simulink model "Three_Stages"  (R2023a)
settings: Solver=FixedStepDiscrete  StartTime=0.0  StopTime=5000  FixedStep=1  RelTol=1e-3
values from neighbouring files (symbols this model uses):
  fw = zeros(16384, 1, 'uint32')    [test.m]
libraries: hdlsllib x27, simulink x27, etargetslib x1
(part 3 of 5)

== system Three_Stages/Subsystem5 ==
  note: // EX -> ID APSR forwarding: CMP/SUBS flags visible to branches in ID
  In2 : Inport
  In5 : Inport  Port=2
  In6 : Inport  Port=3
  In4 : Inport  Port=4
  fwd_n : Inport  Port=5
  fwd_z : Inport  Port=6
  fwd_v : Inport  Port=7
  fwd_c : Inport  Port=8
  alu_n : Inport  Port=9
  alu_z : Inport  Port=10
  alu_v : Inport  Port=11
  alu_c : Inport  Port=12
  Logical Operator : Logic  Inputs=4  AllPortsSameDT=off  OutDataTypeStr=boolean
  Logical Operator1 : Logic  Operator=NOT  AllPortsSameDT=off  OutDataTypeStr=boolean
  Switch{,1..3} (4 alike) : Switch  Criteria=u2 ~= 0  SaturateOnIntegerOverflow=off  InputSameDT=off
  id_instr8 : Outport
  id_instr9 : Outport  Port=2
  id_instr10 : Outport  Port=3
  id_instr11 : Outport  Port=4
  wires:
  alu_z/1 -> Switch/1  "ex_alu_z"
  fwd_z/1 -> Switch/3  "fwd_z"
  In2/1 -> Logical Operator/1  "ex_valid"
  In4/1 -> Logical Operator/2  "ex_s"
  In5/1 -> Logical Operator/3  "ex_cond_ok"
  In6/1 -> Logical Operator1/1  "ex_is_multi_op_raw_nf"
  Logical Operator1/1 -> Logical Operator/4
  Switch/1 -> id_instr8/1  "branch_fwd_z"
  alu_n/1 -> Switch1/1  "ex_alu_n"
  fwd_n/1 -> Switch1/3  "fwd_n"
  Switch1/1 -> id_instr9/1  "branch_fwd_n"
  alu_c/1 -> Switch2/1  "ex_alu_c"
  fwd_c/1 -> Switch2/3  "fwd_c"
  Switch2/1 -> id_instr10/1  "branch_fwd_c"
  alu_v/1 -> Switch3/1  "ex_alu_v"
  fwd_v/1 -> Switch3/3  "fwd_v"
  Switch3/1 -> id_instr11/1  "branch_fwd_v"
  Logical Operator/1 -> Switch3/2, Switch2/2, Switch1/2, Switch/2  "ex_sets_flags"

== system Three_Stages/Subsystem7 ==
  Constant1 : Constant  OutDataTypeStr=boolean
  Constant9 : Constant  OutDataTypeStr=boolean
  Switch1 : Switch  Criteria=u2 ~= 0  SaturateOnIntegerOverflow=off  InputSameDT=off
  Switch13 : Switch  Criteria=u2 ~= 0  SaturateOnIntegerOverflow=off  InputSameDT=off
  rf_we_int : Outport
  tag scope: rf_we_int=global
  wires:
  [mr_rf_we] -> Switch13/2
  Switch1/1 -> Switch13/3
  Constant9/1 -> Switch13/1
  Switch13/1 -> [rf_we_int], rf_we_int/1  "rf_we_int"
  Constant1/1 -> Switch1/1
  [wb_lo_en] -> Switch1/3
  [two_wb_d] -> Switch1/2  "two_wb_d"

== system Three_Stages/Subsystem8 ==
  Switch1 : Switch  Criteria=u2 ~= 0  SaturateOnIntegerOverflow=off  InputSameDT=off
  Switch11 : Switch  Criteria=u2 ~= 0  SaturateOnIntegerOverflow=off  InputSameDT=off
  Switch2 : Switch  Criteria=u2 ~= 0  SaturateOnIntegerOverflow=off  InputSameDT=off
  rf_we_addr_int : Outport
  tag scope: rf_we_addr_int=global
  wires:
  [mr_rf_addr] -> Switch11/1
  [mr_rf_we] -> Switch11/2
  Switch11/1 -> [rf_we_addr_int], rf_we_addr_int/1  "rf_we_addr_int"
  [ex_WB_addr] -> Switch2/3  "ex_WB_addr"
  Switch1/1 -> Switch11/3
  [two_wb_d] -> Switch1/2  "two_wb_d"
  [ex_rd_hi] -> Switch1/1
  Switch2/1 -> Switch1/3
  [ex_two_wb_active] -> Switch2/2  "ex_two_wb_active"
  [ex_rd_lo] -> Switch2/1  "ex_rd_lo"

== system Three_Stages/Subsystem9 ==
  Switch1 : Switch  Criteria=u2 ~= 0  SaturateOnIntegerOverflow=off  InputSameDT=off
  Switch10 : Switch  Criteria=u2 ~= 0  SaturateOnIntegerOverflow=off  InputSameDT=off
  rf_wdata_int : Outport
  wires:
  [mr_rf_wdata] -> Switch10/1
  [mr_rf_we] -> Switch10/2
  Switch10/1 -> rf_wdata_int/1  "rf_wdata_int"
  [rf_wdata] -> Switch1/3  "rf_wdata"
  [two_wb_d] -> Switch1/2  "two_wb_d"
  Switch1/1 -> Switch10/3  "rf_wdata_int"
  [alu_result_hi] -> Switch1/1

== system Three_Stages/i ==
  opcode : Inport
  Constant : Constant  Value=84
  Constant1 : Constant  Value=86
  Constant2 : Constant  Value=58
  Logical Operator : Logic  Operator=OR  AllPortsSameDT=off  OutDataTypeStr=boolean
  Logical Operator1 : Logic  Operator=OR  AllPortsSameDT=off  OutDataTypeStr=boolean
  Relational Operator : RelationalOperator  Operator===  OutDataTypeStr=boolean  RndMeth=Simplest  InputSameDT=off
  Relational Operator1 : RelationalOperator  Operator===  OutDataTypeStr=boolean  RndMeth=Simplest  InputSameDT=off
  Relational Operator2 : RelationalOperator  Operator===  OutDataTypeStr=boolean  RndMeth=Simplest  InputSameDT=off
  Out3 : Outport
  wires:
  Constant/1 -> Relational Operator/2
  Relational Operator/1 -> Logical Operator/1
  Constant1/1 -> Relational Operator1/2
  Relational Operator1/1 -> Logical Operator/2
  Logical Operator/1 -> Logical Operator1/1  "is_adr"
  Constant2/1 -> Relational Operator2/2
  Relational Operator2/1 -> Logical Operator1/2  "is_ldr_lit"
  opcode/1 -> Relational Operator2/1, Relational Operator1/1, Relational Operator/1  "ex_opcode"
  Logical Operator1/1 -> Out3/1  "needs_pc"

== system Three_Stages/id_pc_val2 ==
  In1 : Inport
  In4 : Inport  Port=2
  In5 : Inport  Port=3
  Add : Sum
  Add1 : Sum
  Constant : Constant  Value=4
  Constant1 : Constant  Value=2
  Switch1 : Switch  Criteria=u2 ~= 0  SaturateOnIntegerOverflow=off  InputSameDT=off
  Switch2 : Switch  Criteria=u2 ~= 0  SaturateOnIntegerOverflow=off  InputSameDT=off
  Out1 : Outport
  wires:
  Constant/1 -> Add/2
  Add/1 -> Switch1/1  "pc_plus4"
  Constant1/1 -> Add1/2
  In1/1 -> Switch2/3, Add/1, Add1/1  "pc_addr"
  Add1/1 -> Switch1/3  "pc_plus2"
  In4/1 -> Switch1/2  "pf_width"
  Switch1/1 -> Switch2/1  "pc_inc"
  In5/1 -> Switch2/2  "pf_pop_valid"
  Switch2/1 -> Out1/1  "next_pc"

== system Three_Stages/memory ==
  read_addr : Inport
  write_addr : Inport  Port=2
  read_en : Inport  Port=3
  write_en : Inport  Port=4
  write_data : Inport  Port=5
  instr_addr : Inport  Port=6
  Constant : Constant  Value=fw
  MATLAB Function1 : MATLAB Function  TreatAsAtomicUnit=on
  instr_data : Outport  OutDataTypeStr=uint32
  read_data : Outport  Port=2
  wires:
  [rst_n] -> MATLAB Function1/1(rst_n)
  read_addr/1 -> MATLAB Function1/6(read_addr)
  write_en/1 -> MATLAB Function1/2(write_en)
  read_en/1 -> MATLAB Function1/5(read_en)
  write_data/1 -> MATLAB Function1/4(write_data)
  write_addr/1 -> MATLAB Function1/3(write_addr)
  instr_addr/1 -> MATLAB Function1/7(instr_addr)
  MATLAB Function1/1(read_data) -> read_data/1  "read_data"
  MATLAB Function1/2(instr_data) -> instr_data/1  "instr_data"
  Constant/1 -> MATLAB Function1/8(fw_init)

== system Three_Stages/ALU/REV16 ==
  u : Inport
  Bit Slice2 : hdlsllib/Logic and Bit Operations/Bit Slice  lidx=7  ridx=0
  Bit Slice3 : hdlsllib/Logic and Bit Operations/Bit Slice  lidx=15  ridx=8
  Bit Slice4 : hdlsllib/Logic and Bit Operations/Bit Slice  lidx=23  ridx=16
  Bit Slice5 : hdlsllib/Logic and Bit Operations/Bit Slice  lidx=31  ridx=24
  Bitwise Operator10 : simulink/Logic and Bit Operations/Bitwise Operator  logicop=OR  UseBitMask=off  NumInputPorts=2  BitMask=bin2dec('11011001')  BitMaskRealWorld=Stored Integer
  Bitwise Operator11 : simulink/Logic and Bit Operations/Bitwise Operator  logicop=OR  UseBitMask=off  NumInputPorts=2  BitMask=bin2dec('11011001')  BitMaskRealWorld=Stored Integer
  Bitwise Operator9 : simulink/Logic and Bit Operations/Bitwise Operator  logicop=OR  UseBitMask=off  NumInputPorts=2  BitMask=bin2dec('11011001')  BitMaskRealWorld=Stored Integer
  Shift Arithmetic3 : ArithShift  BitShiftNumber=8  BitShiftDirection=Left
  Shift Arithmetic4 : ArithShift  BitShiftNumber=8  BitShiftDirection=Right
  Shift Arithmetic5 : ArithShift  BitShiftNumber=8  BitShiftDirection=Left
  Shift Arithmetic6 : ArithShift  BitShiftNumber=8  BitShiftDirection=Right
  REV16 : Outport
  wires:
  Bitwise Operator10/1 -> Bitwise Operator11/2
  Shift Arithmetic4/1 -> Bitwise Operator9/2
  Bit Slice3/1 -> Shift Arithmetic4/1
  Bit Slice2/1 -> Shift Arithmetic3/1
  u/1 -> Bit Slice5/1, Bit Slice4/1, Bit Slice3/1, Bit Slice2/1
  Bit Slice4/1 -> Shift Arithmetic5/1
  Shift Arithmetic3/1 -> Bitwise Operator9/1
  Shift Arithmetic6/1 -> Bitwise Operator10/2
  Bit Slice5/1 -> Shift Arithmetic6/1
  Shift Arithmetic5/1 -> Bitwise Operator10/1
  Bitwise Operator9/1 -> Bitwise Operator11/1
  Bitwise Operator11/1 -> REV16/1  "REV16"

== system Three_Stages/ALU/Subsystem ==
  alu_a : Inport
  Bit Slice : hdlsllib/Logic and Bit Operations/Bit Slice  lidx=7  ridx=0
  Bit Slice1 : hdlsllib/Logic and Bit Operations/Bit Slice  lidx=15  ridx=8
  Bitwise Operator11 : simulink/Logic and Bit Operations/Bitwise Operator  logicop=OR  UseBitMask=off  NumInputPorts=2  BitMask=bin2dec('11011001')  BitMaskRealWorld=Stored Integer
  Data Type Conversion1 : DataTypeConversion  OutDataTypeStr=int32  SaturateOnIntegerOverflow=off  RndMeth=Floor
  Data Type Conversion2 : DataTypeConversion  OutDataTypeStr=uint32  SaturateOnIntegerOverflow=off  RndMeth=Floor
  Data Type Conversion6 : DataTypeConversion  OutDataTypeStr=int16  SaturateOnIntegerOverflow=off  RndMeth=Floor
  Shift Arithmetic1 : ArithShift  BitShiftNumber=8  BitShiftDirection=Right
  Shift Arithmetic3 : ArithShift  BitShiftNumber=8  BitShiftDirection=Left
  Out1 : Outport
  wires:
  Bit Slice/1 -> Shift Arithmetic3/1
  Bit Slice1/1 -> Shift Arithmetic1/1
  Shift Arithmetic3/1 -> Bitwise Operator11/1
  Shift Arithmetic1/1 -> Bitwise Operator11/2
  Bitwise Operator11/1 -> Data Type Conversion6/1
  Data Type Conversion6/1 -> Data Type Conversion1/1
  Data Type Conversion1/1 -> Data Type Conversion2/1
  Data Type Conversion2/1 -> Out1/1  "REVSH"
  alu_a/1 -> Bit Slice1/1, Bit Slice/1

== system Three_Stages/ALU/Subsystem1 ==
  alu_a : Inport
  alu_b : Inport  Port=2
  Bitwise Operator1 : simulink/Logic and Bit Operations/Bitwise Operator  logicop=OR  UseBitMask=on  BitMask=0x0000FFFF  BitMaskRealWorld=Stored Integer
  Bitwise Operator2 : simulink/Logic and Bit Operations/Bitwise Operator  logicop=OR  UseBitMask=on  BitMask=0x0000FFFF  BitMaskRealWorld=Stored Integer
  Bitwise Operator3 : simulink/Logic and Bit Operations/Bitwise Operator  logicop=OR  UseBitMask=off  NumInputPorts=2  BitMask=bin2dec('11011001')  BitMaskRealWorld=Stored Integer
  Shift Arithmetic2 : ArithShift  BitShiftNumber=16  BitShiftDirection=Left
  Out1 : Outport
  wires:
  Bitwise Operator3/1 -> Out1/1  "REVSH"
  alu_a/1 -> Bitwise Operator1/1
  Bitwise Operator1/1 -> Bitwise Operator3/1  "lo_keep"
  Bitwise Operator2/1 -> Shift Arithmetic2/1  "imm_lo"
  Shift Arithmetic2/1 -> Bitwise Operator3/2
  alu_b/1 -> Bitwise Operator2/1

== system Three_Stages/ALU/Subsystem2 ==
  In1 : Inport
  In2 : Inport  Port=2
  "alu_acc " : Inport  Port=3
  Add6 : Sum  AccumDataTypeStr=uint64  OutDataTypeStr=uint32
  Data Type Conversion10 : DataTypeConversion  OutDataTypeStr=uint32  SaturateOnIntegerOverflow=off  RndMeth=Floor
  Data Type Conversion9 : DataTypeConversion  OutDataTypeStr=uint64  SaturateOnIntegerOverflow=off  RndMeth=Floor
  Product1 : Product  OutDataTypeStr=uint64
  MLA : Outport
  wires:
  In2/1 -> Product1/2
  Product1/1 -> Add6/1  "prod64"
  Data Type Conversion9/1 -> Add6/2  "acc64"
  Data Type Conversion10/1 -> MLA/1  "MLA"
  "alu_acc "/1 -> Data Type Conversion9/1  "alu_acc"
  Add6/1 -> Data Type Conversion10/1  "sum64"
  In1/1 -> Product1/1

== system Three_Stages/ALU/Subsystem3 ==
  alu_a : Inport
  alu_b : Inport  Port=2
  "alu_acc " : Inport  Port=3
  Add6 : Sum  Inputs=+-  AccumDataTypeStr=uint64  OutDataTypeStr=uint32
  Data Type Conversion10 : DataTypeConversion  OutDataTypeStr=uint32  SaturateOnIntegerOverflow=off  RndMeth=Floor
  Data Type Conversion9 : DataTypeConversion  OutDataTypeStr=uint64  SaturateOnIntegerOverflow=off  RndMeth=Floor
  Product1 : Product  OutDataTypeStr=uint64
  MLS : Outport
  wires:
  alu_b/1 -> Product1/2
  Product1/1 -> Add6/2  "prod64"
  Data Type Conversion9/1 -> Add6/1  "acc64"
  Data Type Conversion10/1 -> MLS/1  "MLA"
  "alu_acc "/1 -> Data Type Conversion9/1  "alu_acc"
  Add6/1 -> Data Type Conversion10/1  "sum64"
  alu_a/1 -> Product1/1

== system Three_Stages/ALU/Subsystem4 ==
  alu_a : Inport
  alu_b : Inport  Port=2
  Bit Slice1 : hdlsllib/Logic and Bit Operations/Bit Slice  lidx=31  ridx=0
  Bit Slice2 : hdlsllib/Logic and Bit Operations/Bit Slice  lidx=63  ridx=32
  Data Type Conversion1 : DataTypeConversion  OutDataTypeStr=uint32  SaturateOnIntegerOverflow=off  RndMeth=Floor
  Data Type Conversion10 : DataTypeConversion  OutDataTypeStr=uint32  SaturateOnIntegerOverflow=off  RndMeth=Floor
  Product1 : Product  OutDataTypeStr=uint64
  MLS : Outport
  MLS1 : Outport  Port=2
  wires:
  alu_b/1 -> Product1/2
  Data Type Conversion10/1 -> MLS/1  "RdLo"
  alu_a/1 -> Product1/1
  Product1/1 -> Bit Slice2/1, Bit Slice1/1  "prod64"
  Bit Slice1/1 -> Data Type Conversion10/1  "result_lo"
  Bit Slice2/1 -> Data Type Conversion1/1  "result_hi"
  Data Type Conversion1/1 -> MLS1/1  "RdHi"

== system Three_Stages/ALU/Subsystem5 ==
  alu_a : Inport
  alu_b : Inport  Port=2
  Bit Slice1 : hdlsllib/Logic and Bit Operations/Bit Slice  lidx=31  ridx=0
  Bit Slice2 : hdlsllib/Logic and Bit Operations/Bit Slice  lidx=63  ridx=32
  Data Type Conversion1 : DataTypeConversion  OutDataTypeStr=uint32  SaturateOnIntegerOverflow=off  RndMeth=Floor
  Data Type Conversion10 : DataTypeConversion  OutDataTypeStr=uint32  SaturateOnIntegerOverflow=off  RndMeth=Floor
  Data Type Conversion2 : DataTypeConversion  OutDataTypeStr=int32  SaturateOnIntegerOverflow=off  RndMeth=Floor
  Data Type Conversion3 : DataTypeConversion  OutDataTypeStr=int32  SaturateOnIntegerOverflow=off  RndMeth=Floor
  Data Type Conversion4 : DataTypeConversion  OutDataTypeStr=int64  SaturateOnIntegerOverflow=off  RndMeth=Floor
  Product1 : Product  OutDataTypeStr=int64
  MLS : Outport
  MLS1 : Outport  Port=2
  wires:
  alu_b/1 -> Data Type Conversion3/1
  Data Type Conversion10/1 -> MLS/1  "RdLo"
  alu_a/1 -> Data Type Conversion2/1
  Data Type Conversion4/1 -> Bit Slice2/1, Bit Slice1/1  "prod_u64"
  Bit Slice1/1 -> Data Type Conversion10/1  "result_lo"
  Bit Slice2/1 -> Data Type Conversion1/1  "result_hi"
  Data Type Conversion1/1 -> MLS1/1  "RdHi"
  Data Type Conversion2/1 -> Product1/1  "a_i32"
  Data Type Conversion3/1 -> Product1/2  "b_i32"
  Product1/1 -> Data Type Conversion4/1  "prod64"

== system Three_Stages/ALU/Subsystem6 ==
  alu_a : Inport
  alu_b : Inport  Port=2
  Constant : Constant  Value=0
  Constant1 : Constant  Value=0
  Data Type Conversion2 : DataTypeConversion  OutDataTypeStr=uint32  SaturateOnIntegerOverflow=off  RndMeth=Floor
  Data Type Conversion3 : DataTypeConversion  OutDataTypeStr=uint32  SaturateOnIntegerOverflow=off  RndMeth=Floor
  Equal : RelationalOperator  Operator===  OutDataTypeStr=boolean  RndMeth=Simplest  InputSameDT=off
  Product1 : Product  Inputs=*/  OutDataTypeStr=uint32
  Switch : Switch  Criteria=u2 ~= 0  SaturateOnIntegerOverflow=off  InputSameDT=off
  MLS : Outport
  wires:
  alu_b/1 -> Equal/1, Data Type Conversion3/1
  alu_a/1 -> Data Type Conversion2/1
  Data Type Conversion2/1 -> Product1/1  "a_i32"
  Data Type Conversion3/1 -> Product1/2  "b_i32"
  Product1/1 -> Switch/3
  Constant/1 -> Equal/2
  Equal/1 -> Switch/2
  Constant1/1 -> Switch/1
  Switch/1 -> MLS/1  "UDIV"

== system Three_Stages/ALU/Subsystem7 ==
  alu_a : Inport
  alu_b : Inport  Port=2
  Constant : Constant  Value=0
  Constant1 : Constant  Value=0
  Data Type Conversion1 : DataTypeConversion  OutDataTypeStr=int32  SaturateOnIntegerOverflow=off
  Data Type Conversion2 : DataTypeConversion  OutDataTypeStr=int32  SaturateOnIntegerOverflow=off  RndMeth=Floor
  Data Type Conversion3 : DataTypeConversion  OutDataTypeStr=int32  SaturateOnIntegerOverflow=off  RndMeth=Floor
  Data Type Conversion4 : DataTypeConversion  OutDataTypeStr=uint32  ConvertRealWorld=Stored Integer (SI)  SaturateOnIntegerOverflow=off  RndMeth=Floor
  Equal : RelationalOperator  Operator===  OutDataTypeStr=boolean  RndMeth=Simplest  InputSameDT=off
  Product1 : Product  Inputs=*/  OutDataTypeStr=double
  Switch : Switch  Criteria=u2 ~= 0  SaturateOnIntegerOverflow=off  InputSameDT=off
  MLS : Outport
  wires:
  alu_b/1 -> Data Type Conversion3/1
  alu_a/1 -> Data Type Conversion2/1
  Data Type Conversion2/1 -> Product1/1  "a_i32"
  Data Type Conversion3/1 -> Equal/2, Product1/2  "b_i32"
  Product1/1 -> Data Type Conversion1/1
  Constant/1 -> Equal/1
  Equal/1 -> Switch/2
  Constant1/1 -> Switch/1
  Switch/1 -> MLS/1  "SDIV"
  Data Type Conversion1/1 -> Data Type Conversion4/1
  Data Type Conversion4/1 -> Switch/3

== system Three_Stages/ALU/Subsystem8 ==
  alu_a : Inport
  "alu_shamt " : Inport  Port=2
  Add : Sum  Inputs=+-
  Bitwise Operator : simulink/Logic and Bit Operations/Bitwise Operator  logicop=OR  UseBitMask=off  NumInputPorts=2  BitMask=bin2dec('11011001')  BitMaskRealWorld=Stored Integer
  Constant3 : Constant  Value=32
  Shift Arithmetic : ArithShift  BitShiftNumberSource=Input port  BitShiftNumber=8  BitShiftDirection=Right
      settings: InputPortMap=u0,p1
  Shift Arithmetic1 : ArithShift  BitShiftNumberSource=Input port  BitShiftNumber=8  BitShiftDirection=Left
      settings: InputPortMap=u0,p1
  MLS1 : Outport
  wires:
  "alu_shamt "/1 -> Add/2, Shift Arithmetic/2  "alu_shamt"
  Constant3/1 -> Add/1
  alu_a/1 -> Shift Arithmetic1/1, Shift Arithmetic/1
  Shift Arithmetic/1 -> Bitwise Operator/1  "sh_r"
  Add/1 -> Shift Arithmetic1/2
  Shift Arithmetic1/1 -> Bitwise Operator/2  "shifted_left"
  Bitwise Operator/1 -> MLS1/1  "ROR"

== system Three_Stages/ALU/Subsystem9 ==
  alu_a : Inport
  "alu_shamt " : Inport  Port=2
  alu_b : Inport  Port=3
  Add : Sum  Inputs=+-  OutDataTypeStr=uint32
  Bitwise Operator : simulink/Logic and Bit Operations/Bitwise Operator  logicop=AND  UseBitMask=off  NumInputPorts=2  BitMask=bin2dec('11011001')  BitMaskRealWorld=Stored Integer
  Constant1 : Constant
  Constant3 : Constant
  Shift Arithmetic : ArithShift  BitShiftNumberSource=Input port  BitShiftNumber=8  BitShiftDirection=Right
      settings: InputPortMap=u0,p1
  Shift Arithmetic1 : ArithShift  BitShiftNumberSource=Input port  BitShiftNumber=8  BitShiftDirection=Left
      settings: InputPortMap=u0,p1
  MLS1 : Outport
  wires:
  "alu_shamt "/1 -> Shift Arithmetic/2  "alu_shamt"
  alu_a/1 -> Shift Arithmetic/1
  Shift Arithmetic/1 -> Bitwise Operator/1  "sh_r"
  Bitwise Operator/1 -> MLS1/1  "UBFX"
  Constant1/1 -> Shift Arithmetic1/1
  Add/1 -> Bitwise Operator/2  "shifted_left"
  Shift Arithmetic1/1 -> Add/1  "shifted_left"
  Constant3/1 -> Add/2
  alu_b/1 -> Shift Arithmetic1/2

== system Three_Stages/Branch_Unit/Subsystem ==
  id_instr : Inport
  id_instr_width : Inport  Port=2
  id_pc : Inport  Port=3
  id_valid : Inport  Port=4
  id_opcode : Inport  Port=5
  id_cond : Inport  Port=6
  id_rm_data : Inport  Port=7
  fwd_z : Inport  Port=8
  fwd_n : Inport  Port=9
  fwd_c : Inport  Port=10
  fwd_v : Inport  Port=11
  MATLAB Function : MATLAB Function  TreatAsAtomicUnit=on
  opcode_sel : Outport
  target_b : Outport  Port=2
  target_bw : Outport  Port=3
  target_bcond : Outport  Port=4
  target_bl : Outport  Port=5
  target_bx : Outport  Port=6
  target_cbz : Outport  Port=7
  cbnz_taken : Outport  Port=8  OutDataTypeStr=boolean
  cbz_taken : Outport  Port=9  OutDataTypeStr=boolean
  cond_pass : Outport  Port=10  OutDataTypeStr=boolean
  wires:
  id_valid/1 -> MATLAB Function/4(id_valid)
  MATLAB Function/8(target_cbz) -> target_cbz/1
  MATLAB Function/7(target_bx) -> target_bx/1
  id_instr/1 -> MATLAB Function/1(id_instr)
  MATLAB Function/1(cond_pass) -> cond_pass/1
  MATLAB Function/4(target_bw) -> target_bw/1
  fwd_v/1 -> MATLAB Function/11(fwd_v)
  id_pc/1 -> MATLAB Function/3(id_pc)
  id_rm_data/1 -> MATLAB Function/7(id_rm_data)
  MATLAB Function/9(cbz_taken) -> cbz_taken/1
  MATLAB Function/5(target_bcond) -> target_bcond/1
  id_opcode/1 -> MATLAB Function/5(id_opcode)
  id_cond/1 -> MATLAB Function/6(id_cond)
  fwd_n/1 -> MATLAB Function/9(fwd_n)
  fwd_z/1 -> MATLAB Function/8(fwd_z)
  MATLAB Function/3(target_b) -> target_b/1
  fwd_c/1 -> MATLAB Function/10(fwd_c)
  MATLAB Function/2(opcode_sel) -> opcode_sel/1
  MATLAB Function/10(cbnz_taken) -> cbnz_taken/1
  id_instr_width/1 -> MATLAB Function/2(id_instr_width)
  MATLAB Function/6(target_bl) -> target_bl/1

== system Three_Stages/Forward_Unit/Forwarding source 1: EX -> ID (same cycle) ==
  Logical Operator1 : Logic  AllPortsSameDT=off  OutDataTypeStr=boolean
  Logical Operator11 : Logic  Inputs=4  AllPortsSameDT=off  OutDataTypeStr=boolean
  Logical Operator2 : Logic  AllPortsSameDT=off  OutDataTypeStr=boolean
  Logical Operator3 : Logic  Inputs=4  AllPortsSameDT=off  OutDataTypeStr=boolean
  Logical Operator4 : Logic  Operator=NOT  AllPortsSameDT=off  OutDataTypeStr=boolean
  Logical Operator5 : Logic  Operator=NOT  AllPortsSameDT=off  OutDataTypeStr=boolean
  Relational Operator : RelationalOperator  Operator===  OutDataTypeStr=boolean  RndMeth=Simplest  InputSameDT=off
  Relational Operator1 : RelationalOperator  Operator===  OutDataTypeStr=boolean  RndMeth=Simplest  InputSameDT=off
  Out1 : Outport
  Out2 : Outport  Port=2
  wires:
  [ex_WB_en_eff] -> Logical Operator11/2
  [id_read_addr_1] -> Relational Operator/2
  [ex_valid_eff] -> Logical Operator11/1
  Logical Operator11/1 -> Out1/1  "fwd_data_1_hit"
  [id_read_en_1] -> Logical Operator1/1
  [ex_WB_addr] -> Relational Operator/1
  Logical Operator1/1 -> Logical Operator11/4
  Relational Operator/1 -> Logical Operator1/2
  [id_read_en_2] -> Logical Operator2/1
  [ex_WB_addr] -> Relational Operator1/1
  [ex_valid_eff] -> Logical Operator3/1
  Logical Operator3/1 -> Out2/1  "fwd_data_2_hit"
  Logical Operator2/1 -> Logical Operator3/4
  Relational Operator1/1 -> Logical Operator2/2
  [id_read_addr_2] -> Relational Operator1/2
  [ex_WB_en_eff] -> Logical Operator3/2
  [ex_is_multi_op] -> Logical Operator4/1
  [ex_is_multi_op] -> Logical Operator5/1
  Logical Operator4/1 -> Logical Operator11/3
  Logical Operator5/1 -> Logical Operator3/3

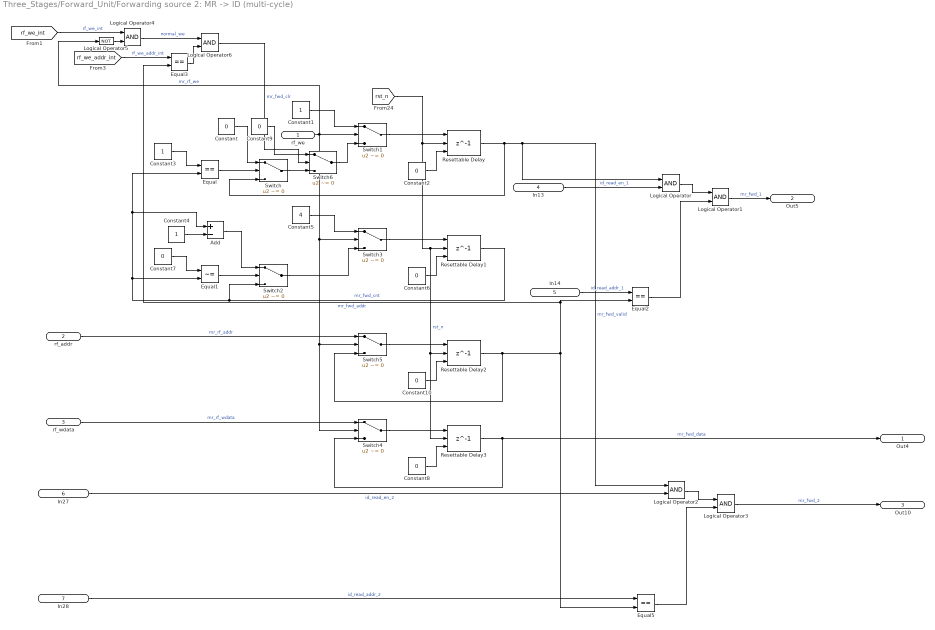
== system Three_Stages/Forward_Unit/Forwarding source 2: MR -> ID (multi-cycle) ==
  rf_we : Inport
  rf_addr : Inport  Port=2
  rf_wdata : Inport  Port=3
  In13 : Inport  Port=4
  In14 : Inport  Port=5
  In27 : Inport  Port=6
  In28 : Inport  Port=7
  Add : Sum  Inputs=+-
  Constant{,2,6..7,9} (5 alike) : Constant  Value=0
  Constant1 : Constant
  Constant10 : Constant  Value=0  OutDataTypeStr=uint32
  Constant3 : Constant
  Constant4 : Constant
  Constant5 : Constant  Value=4  OutDataTypeStr=uint8
  Constant8 : Constant  Value=0  OutDataTypeStr=uint32
  Equal{,2..3,5} (4 alike) : RelationalOperator  Operator===  OutDataTypeStr=boolean  RndMeth=Simplest  InputSameDT=off
  Equal1 : RelationalOperator  Operator=~=  OutDataTypeStr=boolean  RndMeth=Simplest  InputSameDT=off
  Logical Operator{,1..4,6} (6 alike) : Logic  AllPortsSameDT=off  OutDataTypeStr=boolean
  Logical Operator5 : Logic  Operator=NOT  AllPortsSameDT=off  OutDataTypeStr=boolean
  Resettable Delay{,1..3} (4 alike) : Delay  DelayLength=1  InitialConditionSource=Input port  ExternalReset=Falling
      settings: InputPortMap=u0,r5,p4
  Switch{,1..3,6} (5 alike) : Switch  Criteria=u2 ~= 0  SaturateOnIntegerOverflow=off  InputSameDT=off
  Switch4 : Switch  Criteria=u2 ~= 0  OutDataTypeStr=uint32  SaturateOnIntegerOverflow=off  InputSameDT=off
  Switch5 : Switch  Criteria=u2 ~= 0  OutDataTypeStr=uint32  SaturateOnIntegerOverflow=off  InputSameDT=off
  Out4 : Outport
  Out5 : Outport  Port=2
  Out10 : Outport  Port=3
  wires:
  Constant/1 -> Switch/1
  Switch/1 -> Switch6/3
  Constant1/1 -> Switch1/1
  Switch1/1 -> Resettable Delay/1
  Constant2/1 -> Resettable Delay/3
  Equal/1 -> Switch/2
  Constant3/1 -> Equal/1
  Constant7/1 -> Equal1/1
  Add/1 -> Switch2/1
  Equal1/1 -> Switch2/2
  Constant6/1 -> Resettable Delay1/3
  Switch2/1 -> Switch3/3
  Switch3/1 -> Resettable Delay1/1
  Constant5/1 -> Switch3/1
  Constant4/1 -> Add/2
  Switch5/1 -> Resettable Delay2/1
  Constant10/1 -> Resettable Delay2/3
  Switch4/1 -> Resettable Delay3/1
  Resettable Delay3/1 -> Switch4/3, Out4/1  "mr_fwd_data"
  Constant8/1 -> Resettable Delay3/3
  In13/1 -> Logical Operator/2  "id_read_en_1"
  Logical Operator/1 -> Logical Operator1/1
  Logical Operator1/1 -> Out5/1  "mr_fwd_1"
  Equal2/1 -> Logical Operator1/2
  In14/1 -> Equal2/1  "id_read_addr_1"
  In27/1 -> Logical Operator2/2  "id_read_en_2"
  Logical Operator3/1 -> Out10/1  "mr_fwd_2"
  In28/1 -> Equal5/1  "id_read_addr_2"
  [rst_n] -> Resettable Delay/2, Resettable Delay3/2, Resettable Delay2/2, Resettable Delay1/2  "rst_n"
  rf_wdata/1 -> Switch4/1  "mr_rf_wdata"
  Logical Operator2/1 -> Logical Operator3/1
  Resettable Delay/1 -> Switch/3, Logical Operator/1, Logical Operator2/1  "mr_fwd_valid"
  rf_addr/1 -> Switch5/1  "mr_rf_addr"
  Resettable Delay1/1 -> Equal/2, Add/1, Equal1/2, Switch2/3  "mr_fwd_cnt"
  Equal5/1 -> Logical Operator3/2
  Logical Operator4/1 -> Logical Operator6/1  "normal_we"
  rf_we/1 -> Logical Operator5/1, Switch4/2, Switch5/2, Switch3/2, Switch1/2  "mr_rf_we"
  [rf_we_int] -> Logical Operator4/1  "rf_we_int"
  Logical Operator5/1 -> Logical Operator4/2
  Logical Operator6/1 -> Switch6/2  "mr_fwd_clr"
  Equal3/1 -> Logical Operator6/2
  [rf_we_addr_int] -> Equal3/1  "rf_we_addr_int"
  Resettable Delay2/1 -> Switch5/3, Equal3/2, Equal2/2, Equal5/2  "mr_fwd_addr"
  Switch6/1 -> Switch1/3
  Constant9/1 -> Switch6/1

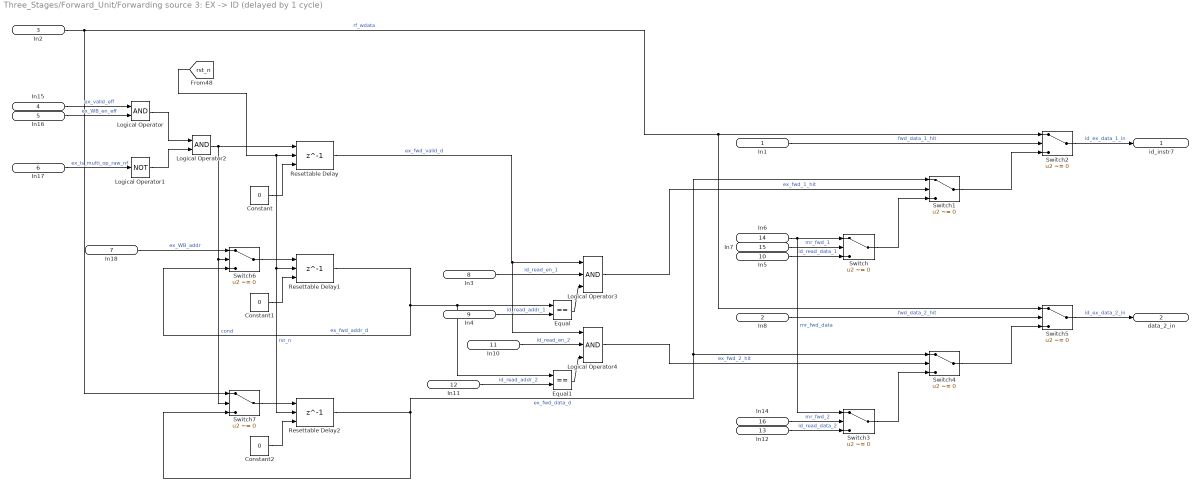
== system Three_Stages/Forward_Unit/Forwarding source 3: EX -> ID (delayed by 1 cycle) ==
  In1 : Inport
  In8 : Inport  Port=2
  In2 : Inport  Port=3
  In15 : Inport  Port=4
  In16 : Inport  Port=5
  In17 : Inport  Port=6
  In18 : Inport  Port=7
  In3 : Inport  Port=8
  In4 : Inport  Port=9
  In5 : Inport  Port=10
  In10 : Inport  Port=11
  In11 : Inport  Port=12
  In12 : Inport  Port=13
  In6 : Inport  Port=14
  In7 : Inport  Port=15
  In14 : Inport  Port=16
  Constant : Constant  Value=0  OutDataTypeStr=boolean
  Constant1 : Constant  Value=0  OutDataTypeStr=uint8
  Constant2 : Constant  Value=0
  Equal : RelationalOperator  Operator===  OutDataTypeStr=boolean  RndMeth=Simplest  InputSameDT=off
  Equal1 : RelationalOperator  Operator===  OutDataTypeStr=boolean  RndMeth=Simplest  InputSameDT=off
  Logical Operator : Logic  AllPortsSameDT=off  OutDataTypeStr=boolean
  Logical Operator1 : Logic  Operator=NOT  AllPortsSameDT=off  OutDataTypeStr=boolean
  Logical Operator2 : Logic  AllPortsSameDT=off  OutDataTypeStr=boolean
  Logical Operator3 : Logic  Inputs=3  AllPortsSameDT=off  OutDataTypeStr=boolean
  Logical Operator4 : Logic  Inputs=3  AllPortsSameDT=off  OutDataTypeStr=boolean
  Resettable Delay : Delay  DelayLength=1  InitialConditionSource=Input port  ExternalReset=Falling
      settings: InputPortMap=u0,r5,p4
  Resettable Delay1 : Delay  DelayLength=1  InitialConditionSource=Input port  ExternalReset=Falling
      settings: InputPortMap=u0,r5,p4
  Resettable Delay2 : Delay  DelayLength=1  InitialConditionSource=Input port  ExternalReset=Falling
      settings: InputPortMap=u0,r5,p4
  Switch{,1..7} (8 alike) : Switch  Criteria=u2 ~= 0  SaturateOnIntegerOverflow=off  InputSameDT=off
  id_instr7 : Outport
  data_2_in : Outport  Port=2
  wires:
  In1/1 -> Switch2/2  "fwd_data_1_hit"
  Switch1/1 -> Switch2/3
  Switch/1 -> Switch1/3
  Switch2/1 -> id_instr7/1  "id_ex_data_1_in"
  Resettable Delay2/1 -> Switch7/3, Switch1/1, Switch4/1  "ex_fwd_data_d"
  In5/1 -> Switch/3  "id_read_data_1"
  In7/1 -> Switch/2  "mr_fwd_1"
  Switch4/1 -> Switch5/3
  In2/1 -> Switch5/1, Switch2/1, Switch7/1  "rf_wdata"
  In6/1 -> Switch3/1, Switch/1  "mr_fwd_data"
  In14/1 -> Switch3/2  "mr_fwd_2"
  In8/1 -> Switch5/2  "fwd_data_2_hit"
  In12/1 -> Switch3/3  "id_read_data_2"
  Switch3/1 -> Switch4/3
  Switch5/1 -> data_2_in/1  "id_ex_data_2_in"
  In15/1 -> Logical Operator/1  "ex_valid_eff"
  In16/1 -> Logical Operator/2  "ex_WB_en_eff"
  In17/1 -> Logical Operator1/1  "ex_is_multi_op_raw_nf"
  Logical Operator/1 -> Logical Operator2/1
  Logical Operator1/1 -> Logical Operator2/2
  Constant/1 -> Resettable Delay/3
  In18/1 -> Switch6/1  "ex_WB_addr"
  Switch6/1 -> Resettable Delay1/1
  Constant1/1 -> Resettable Delay1/3
  [rst_n] -> Resettable Delay2/2, Resettable Delay1/2, Resettable Delay/2  "rst_n"
  Logical Operator2/1 -> Resettable Delay/1, Switch7/2, Switch6/2  "cond"
  Switch7/1 -> Resettable Delay2/1
  Constant2/1 -> Resettable Delay2/3
  In3/1 -> Logical Operator3/2  "id_read_en_1"
  In4/1 -> Equal/2  "id_read_addr_1"
  Equal/1 -> Logical Operator3/3
  Logical Operator3/1 -> Switch1/2  "ex_fwd_1_hit"
  In10/1 -> Logical Operator4/2  "id_read_en_2"
  Equal1/1 -> Logical Operator4/3
  Logical Operator4/1 -> Switch4/2  "ex_fwd_2_hit"
  In11/1 -> Equal1/2  "id_read_addr_2"
  Resettable Delay/1 -> Logical Operator4/1, Logical Operator3/1  "ex_fwd_valid_d"
  Resettable Delay1/1 -> Equal1/1, Equal/1, Switch6/3  "ex_fwd_addr_d"

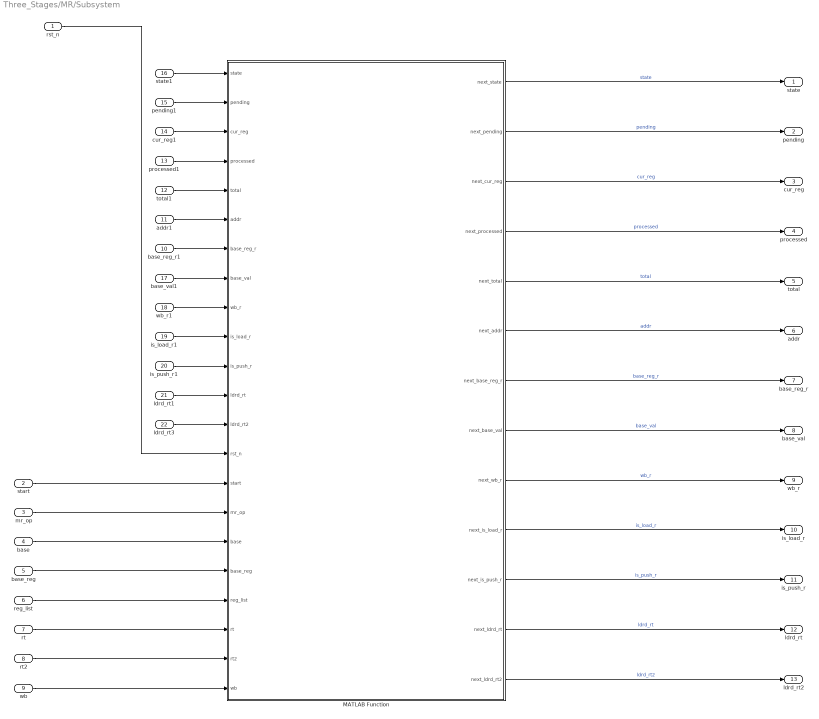
== system Three_Stages/MR/Subsystem ==
  rst_n : Inport
  start : Inport  Port=2
  mr_op : Inport  Port=3
  base : Inport  Port=4
  base_reg : Inport  Port=5
  reg_list : Inport  Port=6
  rt : Inport  Port=7
  rt2 : Inport  Port=8
  wb : Inport  Port=9
  base_reg_r1 : Inport  Port=10
  addr1 : Inport  Port=11
  total1 : Inport  Port=12
  processed1 : Inport  Port=13
  cur_reg1 : Inport  Port=14
  pending1 : Inport  Port=15
  state1 : Inport  Port=16
  base_val1 : Inport  Port=17
  wb_r1 : Inport  Port=18
  is_load_r1 : Inport  Port=19
  is_push_r1 : Inport  Port=20
  ldrd_rt1 : Inport  Port=21
  ldrd_rt3 : Inport  Port=22
  MATLAB Function : MATLAB Function  TreatAsAtomicUnit=on
  state : Outport
  pending : Outport  Port=2
  cur_reg : Outport  Port=3
  processed : Outport  Port=4
  total : Outport  Port=5
  addr : Outport  Port=6
  base_reg_r : Outport  Port=7
  base_val : Outport  Port=8
  wb_r : Outport  Port=9
  is_load_r : Outport  Port=10
  is_push_r : Outport  Port=11
  ldrd_rt : Outport  Port=12
  ldrd_rt2 : Outport  Port=13
  wires:
  base_reg_r1/1 -> MATLAB Function/7(base_reg_r)
  pending1/1 -> MATLAB Function/2(pending)
  wb/1 -> MATLAB Function/22(wb)
  MATLAB Function/4(next_processed) -> processed/1  "processed"
  MATLAB Function/11(next_is_push_r) -> is_push_r/1  "is_push_r"
  addr1/1 -> MATLAB Function/6(addr)
  base_reg/1 -> MATLAB Function/18(base_reg)
  MATLAB Function/9(next_wb_r) -> wb_r/1  "wb_r"
  state1/1 -> MATLAB Function/1(state)
  rt2/1 -> MATLAB Function/21(rt2)
  base_val1/1 -> MATLAB Function/8(base_val)
  is_push_r1/1 -> MATLAB Function/11(is_push_r)
  MATLAB Function/7(next_base_reg_r) -> base_reg_r/1  "base_reg_r"
  total1/1 -> MATLAB Function/5(total)
  MATLAB Function/2(next_pending) -> pending/1  "pending"
  cur_reg1/1 -> MATLAB Function/3(cur_reg)
  is_load_r1/1 -> MATLAB Function/10(is_load_r)
  base/1 -> MATLAB Function/17(base)
  rst_n/1 -> MATLAB Function/14(rst_n)
  MATLAB Function/5(next_total) -> total/1  "total"
  processed1/1 -> MATLAB Function/4(processed)
  MATLAB Function/12(next_ldrd_rt) -> ldrd_rt/1  "ldrd_rt"
  MATLAB Function/8(next_base_val) -> base_val/1  "base_val"
  start/1 -> MATLAB Function/15(start)
  MATLAB Function/3(next_cur_reg) -> cur_reg/1  "cur_reg"
  MATLAB Function/10(next_is_load_r) -> is_load_r/1  "is_load_r"
  MATLAB Function/1(next_state) -> state/1  "state"
  wb_r1/1 -> MATLAB Function/9(wb_r)
  ldrd_rt3/1 -> MATLAB Function/13(ldrd_rt2)
  rt/1 -> MATLAB Function/20(rt)
  MATLAB Function/13(next_ldrd_rt2) -> ldrd_rt2/1  "ldrd_rt2"
  MATLAB Function/6(next_addr) -> addr/1  "addr"
  reg_list/1 -> MATLAB Function/19(reg_list)
  ldrd_rt1/1 -> MATLAB Function/12(ldrd_rt)
  mr_op/1 -> MATLAB Function/16(mr_op)

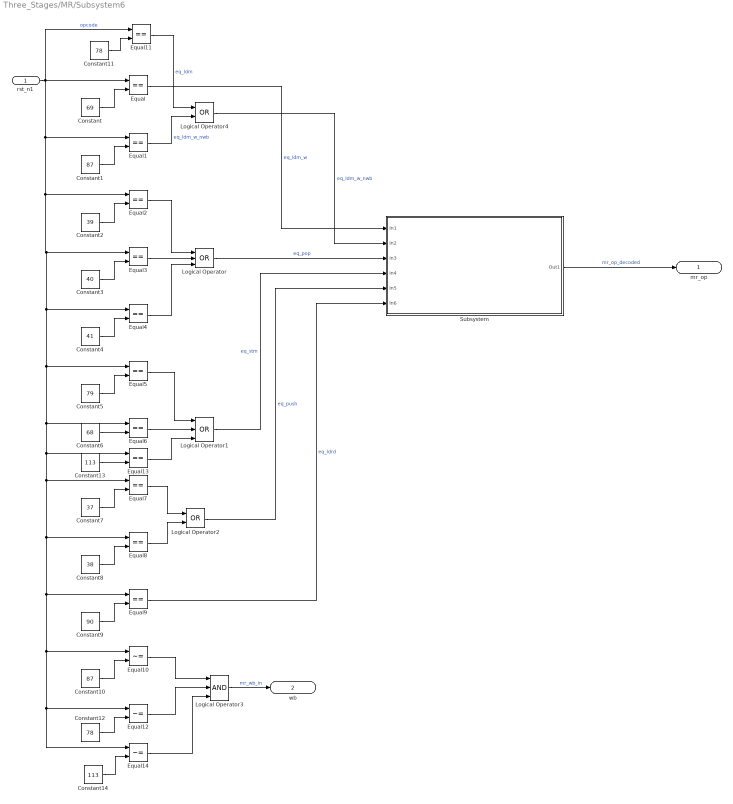
== system Three_Stages/MR/Subsystem6 ==
  rst_n1 : Inport
  Constant : Constant  Value=69
  Constant1 : Constant  Value=87
  Constant10 : Constant  Value=87
  Constant11 : Constant  Value=78
  Constant12 : Constant  Value=78
  Constant13 : Constant  Value=113
  Constant14 : Constant  Value=113
  Constant2 : Constant  Value=39
  Constant3 : Constant  Value=40
  Constant4 : Constant  Value=41
  Constant5 : Constant  Value=79
  Constant6 : Constant  Value=68
  Constant7 : Constant  Value=37
  Constant8 : Constant  Value=38
  Constant9 : Constant  Value=90
  Equal{,1..9,11,13} (12 alike) : RelationalOperator  Operator===  OutDataTypeStr=boolean  RndMeth=Simplest  InputSameDT=off
  Equal10 : RelationalOperator  Operator=~=  OutDataTypeStr=boolean  RndMeth=Simplest  InputSameDT=off
  Equal12 : RelationalOperator  Operator=~=  OutDataTypeStr=boolean  RndMeth=Simplest  InputSameDT=off
  Equal14 : RelationalOperator  Operator=~=  OutDataTypeStr=boolean  RndMeth=Simplest  InputSameDT=off
  Logical Operator : Logic  Operator=OR  Inputs=3  AllPortsSameDT=off  OutDataTypeStr=boolean
  Logical Operator1 : Logic  Operator=OR  Inputs=3  AllPortsSameDT=off  OutDataTypeStr=boolean
  Logical Operator2 : Logic  Operator=OR  AllPortsSameDT=off  OutDataTypeStr=boolean
  Logical Operator3 : Logic  Inputs=3  AllPortsSameDT=off  OutDataTypeStr=boolean
  Logical Operator4 : Logic  Operator=OR  AllPortsSameDT=off  OutDataTypeStr=boolean
  Subsystem : Subsystem
  mr_op : Outport  OutDataTypeStr=uint8
  wb : Outport  Port=2
  wires:
  Constant/1 -> Equal/2
  Constant1/1 -> Equal1/2
  Constant2/1 -> Equal2/2
  Constant3/1 -> Equal3/2
  Constant5/1 -> Equal5/2
  Constant4/1 -> Equal4/2
  Constant8/1 -> Equal8/2
  Constant7/1 -> Equal7/2
  Constant6/1 -> Equal6/2
  Constant9/1 -> Equal9/2
  rst_n1/1 -> Equal11/1, Equal/1, Equal14/1, Equal12/1, Equal10/1, Equal9/1, Equal8/1, Equal7/1, Equal13/1, Equal6/1, Equal5/1, Equal4/1, Equal3/1, Equal2/1, Equal1/1  "opcode"
  Constant10/1 -> Equal10/2
  Equal/1 -> Subsystem/1(In1)  "eq_ldm_w"
  Logical Operator4/1 -> Subsystem/2(In2)  "eq_ldm_w_nwb"
  Equal2/1 -> Logical Operator/1
  Equal3/1 -> Logical Operator/2
  Equal4/1 -> Logical Operator/3
  Logical Operator/1 -> Subsystem/3(In3)  "eq_pop"
  Equal5/1 -> Logical Operator1/1
  Equal6/1 -> Logical Operator1/2
  Logical Operator1/1 -> Subsystem/4(In4)  "eq_stm"
  Equal7/1 -> Logical Operator2/1
  Equal8/1 -> Logical Operator2/2
  Logical Operator2/1 -> Subsystem/5(In5)  "eq_push"
  Equal9/1 -> Subsystem/6(In6)  "eq_ldrd"
  Equal10/1 -> Logical Operator3/1
  Subsystem/1(Out1) -> mr_op/1  "mr_op_decoded"
  Constant11/1 -> Equal11/2
  Equal12/1 -> Logical Operator3/2
  Constant12/1 -> Equal12/2
  Logical Operator3/1 -> wb/1  "mr_wb_in"
  Equal11/1 -> Logical Operator4/1  "eq_ldm"
  Equal1/1 -> Logical Operator4/2  "eq_ldm_w_nwb"
  Equal13/1 -> Logical Operator1/3
  Constant13/1 -> Equal13/2
  Constant14/1 -> Equal14/2
  Equal14/1 -> Logical Operator3/3

== system Three_Stages/Prefetch_Unit/Subsystem ==
  instr_data : Inport
  flush : Inport  Port=2
  flush_target : Inport  Port=3
  stall : Inport  Port=4
  count : Inport  Port=5
  rd_ptr : Inport  Port=6
  wr_ptr : Inport  Port=7
  fifo_mem : Inport  Port=8
  fetch_pc : Inport  Port=9
  instr : Inport  Port=10
  instr_width : Inport  Port=11
  pop_valid : Inport  Port=12
  MATLAB Function : MATLAB Function  TreatAsAtomicUnit=on
  next_fifo_mem : Outport  OutDataTypeStr=uint16
  next_wr_ptr : Outport  Port=2  OutDataTypeStr=uint8
  next_rd_ptr : Outport  Port=3  OutDataTypeStr=uint8
  next_count : Outport  Port=4  OutDataTypeStr=uint8
  next_fetch_pc : Outport  Port=5  OutDataTypeStr=uint32
  next_instr : Outport  Port=6  OutDataTypeStr=uint32
  next_instr_width : Outport  Port=7  OutDataTypeStr=boolean
  next_pop_valid : Outport  Port=8
  wires:
  MATLAB Function/4(next_count) -> next_count/1
  MATLAB Function/1(next_fifo_mem) -> next_fifo_mem/1
  MATLAB Function/3(next_rd_ptr) -> next_rd_ptr/1
  MATLAB Function/5(next_fetch_pc) -> next_fetch_pc/1
  MATLAB Function/6(next_instr) -> next_instr/1
  MATLAB Function/2(next_wr_ptr) -> next_wr_ptr/1
  flush/1 -> MATLAB Function/10(flush)
  MATLAB Function/7(next_instr_width) -> next_instr_width/1
  MATLAB Function/8(next_pop_valid) -> next_pop_valid/1
  count/1 -> MATLAB Function/4(count)
  fifo_mem/1 -> MATLAB Function/1(fifo_mem)
  instr_width/1 -> MATLAB Function/7(instr_width)
  pop_valid/1 -> MATLAB Function/8(pop_valid)
  wr_ptr/1 -> MATLAB Function/2(wr_ptr)
  rd_ptr/1 -> MATLAB Function/3(rd_ptr)
  instr/1 -> MATLAB Function/6(instr)
  fetch_pc/1 -> MATLAB Function/5(fetch_pc)
  flush_target/1 -> MATLAB Function/11(flush_target)
  instr_data/1 -> MATLAB Function/9(instr_data)
  stall/1 -> MATLAB Function/12(stall)

== system Three_Stages/STRB_STRH/Subsystem ==
  ex_alu_result : Inport
  first_read_cond : Inport  Port=2
  Constant8 : Constant  Value=0  OutDataTypeStr=uint8
  Resettable Delay1 : Delay  DelayLength=1  InitialConditionSource=Input port  ExternalReset=Falling
      settings: InputPortMap=u0,r5,p4
  Switch3 : Switch  Criteria=u2 ~= 0  SaturateOnIntegerOverflow=off  InputSameDT=off
  saved_addr : Outport
  wires:
  first_read_cond/1 -> Switch3/2
  Resettable Delay1/1 -> saved_addr/1, Switch3/3  "saved_addr"
  Constant8/1 -> Resettable Delay1/3
  ex_alu_result/1 -> Switch3/1
  [rst_n] -> Resettable Delay1/2
  Switch3/1 -> Resettable Delay1/1

== system Three_Stages/STRB_STRH/Subsystem1 ==
  ex_data_2 : Inport
  first_read_cond : Inport  Port=2
  Constant8 : Constant  Value=0  OutDataTypeStr=uint8
  Resettable Delay1 : Delay  DelayLength=1  InitialConditionSource=Input port  ExternalReset=Falling
      settings: InputPortMap=u0,r5,p4
  Switch3 : Switch  Criteria=u2 ~= 0  SaturateOnIntegerOverflow=off  InputSameDT=off
  saved_rs2 : Outport
  wires:
  first_read_cond/1 -> Switch3/2
  Resettable Delay1/1 -> saved_rs2/1, Switch3/3
  Constant8/1 -> Resettable Delay1/3
  ex_data_2/1 -> Switch3/1
  [rst_n] -> Resettable Delay1/2
  Switch3/1 -> Resettable Delay1/1

== system Three_Stages/STRB_STRH/Subsystem2 ==
  is_strb : Inport
  first_read_cond : Inport  Port=2
  Constant8 : Constant  Value=0  OutDataTypeStr=uint8
  Resettable Delay1 : Delay  DelayLength=1  InitialConditionSource=Input port  ExternalReset=Falling
      settings: InputPortMap=u0,r5,p4
  Switch3 : Switch  Criteria=u2 ~= 0  SaturateOnIntegerOverflow=off  InputSameDT=off
  saved_is_strb : Outport
  wires:
  first_read_cond/1 -> Switch3/2
  Resettable Delay1/1 -> saved_is_strb/1, Switch3/3
  Constant8/1 -> Resettable Delay1/3
  is_strb/1 -> Switch3/1
  [rst_n] -> Resettable Delay1/2
  Switch3/1 -> Resettable Delay1/1

== system Three_Stages/STRB_STRH/Subsystem3 ==
  is_strh : Inport
  first_read_cond : Inport  Port=2
  Constant8 : Constant  Value=0  OutDataTypeStr=uint8
  Resettable Delay1 : Delay  DelayLength=1  InitialConditionSource=Input port  ExternalReset=Falling
      settings: InputPortMap=u0,r5,p4
  Switch3 : Switch  Criteria=u2 ~= 0  SaturateOnIntegerOverflow=off  InputSameDT=off
  saved_is_strh : Outport
  wires:
  first_read_cond/1 -> Switch3/2
  Resettable Delay1/1 -> saved_is_strh/1, Switch3/3
  Constant8/1 -> Resettable Delay1/3
  is_strh/1 -> Switch3/1
  [rst_n] -> Resettable Delay1/2
  Switch3/1 -> Resettable Delay1/1

== system Three_Stages/STRB_STRH/Subsystem4 ==
  mem_rdata : Inport
  first_read_cond : Inport  Port=2
  Constant8 : Constant  Value=0  OutDataTypeStr=uint8
  Resettable Delay1 : Delay  DelayLength=1  InitialConditionSource=Input port  ExternalReset=Falling
      settings: InputPortMap=u0,r5,p4
  Switch3 : Switch  Criteria=u2 ~= 0  SaturateOnIntegerOverflow=off  InputSameDT=off
  saved_rdata : Outport
  wires:
  first_read_cond/1 -> Switch3/2
  Resettable Delay1/1 -> saved_rdata/1, Switch3/3
  Constant8/1 -> Resettable Delay1/3
  mem_rdata/1 -> Switch3/1
  [rst_n] -> Resettable Delay1/2
  Switch3/1 -> Resettable Delay1/1

== system Three_Stages/STRB_STRH/Subsystem6 ==
  is_strd : Inport
  first_read_cond : Inport  Port=2
  Constant8 : Constant  Value=0  OutDataTypeStr=uint8
  Resettable Delay1 : Delay  DelayLength=1  InitialConditionSource=Input port  ExternalReset=Falling
      settings: InputPortMap=u0,r5,p4
  Switch3 : Switch  Criteria=u2 ~= 0  SaturateOnIntegerOverflow=off  InputSameDT=off
  saved_is_strd : Outport
  wires:
  first_read_cond/1 -> Switch3/2
  Resettable Delay1/1 -> saved_is_strd/1, Switch3/3
  Constant8/1 -> Resettable Delay1/3
  is_strd/1 -> Switch3/1
  [rst_n] -> Resettable Delay1/2
  Switch3/1 -> Resettable Delay1/1

== system Three_Stages/Subsystem2/Subsystem ==
  opcode : Inport
  stall : Inport  Port=2
  instr : Inport  Port=3
  instr_valid : Inport  Port=4
  rst_n : Inport  Port=5
  it_cond_reg : Inport  Port=6
  it_count_reg : Inport  Port=7
  it_active_reg : Inport  Port=8
  MATLAB Function2 : MATLAB Function  TreatAsAtomicUnit=on
  it_cond_next : Outport
  it_count_next : Outport  Port=2  OutDataTypeStr=uint8
  it_active_next : Outport  Port=3  OutDataTypeStr=boolean
  wires:
  rst_n/1 -> MATLAB Function2/1(rst_n)
  stall/1 -> MATLAB Function2/2(stall)
  it_active_reg/1 -> MATLAB Function2/8(it_active_reg)
  MATLAB Function2/1(it_cond_next) -> it_cond_next/1
  instr_valid/1 -> MATLAB Function2/4(instr_valid)
  it_count_reg/1 -> MATLAB Function2/7(it_count_reg)
  MATLAB Function2/2(it_count_next) -> it_count_next/1
  MATLAB Function2/3(it_active_next) -> it_active_next/1
  it_cond_reg/1 -> MATLAB Function2/6(it_cond_reg)
  opcode/1 -> MATLAB Function2/5(opcode)
  instr/1 -> MATLAB Function2/3(instr)

== system Three_Stages/Subsystem2/Subsystem1 ==
  instr : Inport
  instr_width : Inport  Port=2
  instr_valid : Inport  Port=3
  it_cond_reg : Inport  Port=4  OutDataTypeStr=uint8
  it_active_reg : Inport  Port=5
  MATLAB Function1 : MATLAB Function  TreatAsAtomicUnit=on
  opcode : Outport
  s : Outport  Port=2
  cond : Outport  Port=3
  valid : Outport  Port=4
  rd : Outport  Port=5
  rn : Outport  Port=6
  rm : Outport  Port=7
  imm24 : Outport  Port=8
  imm32 : Outport  Port=9
  read_addr_1 : Outport  Port=10
  read_en_1 : Outport  Port=11
  read_addr_2 : Outport  Port=12
  read_en_2 : Outport  Port=13
  write_en : Outport  Port=14
  alu_op : Outport  Port=15
  alu_src_b : Outport  Port=16
  alu_use_carry : Outport  Port=17
  alu_shamt : Outport  Port=18
  alu_shift_type : Outport  Port=19
  reg_list : Outport  Port=20
  ra : Outport  Port=21
  ra_valid : Outport  Port=22
  rd_lo : Outport  Port=23
  rd_hi : Outport  Port=24
  two_wb : Outport  Port=25
  wires:
  MATLAB Function1/24(alu_shift_type) -> alu_shift_type/1
  MATLAB Function1/22(alu_use_carry) -> alu_use_carry/1
  MATLAB Function1/1(opcode) -> opcode/1
  MATLAB Function1/3(cond) -> cond/1
  it_cond_reg/1 -> MATLAB Function1/4(it_cond_reg)
  MATLAB Function1/25(reg_list) -> reg_list/1
  MATLAB Function1/2(s) -> s/1
  instr_valid/1 -> MATLAB Function1/3(instr_valid)
  MATLAB Function1/16(read_en_1) -> read_en_1/1
  instr/1 -> MATLAB Function1/1(instr)
  MATLAB Function1/23(alu_shamt) -> alu_shamt/1
  instr_width/1 -> MATLAB Function1/2(instr_width)
  it_active_reg/1 -> MATLAB Function1/5(it_active_reg)
  MATLAB Function1/5(rd) -> rd/1
  MATLAB Function1/4(valid) -> valid/1
  MATLAB Function1/7(rm) -> rm/1
  MATLAB Function1/6(rn) -> rn/1
  MATLAB Function1/13(imm24) -> imm24/1
  MATLAB Function1/17(read_addr_2) -> read_addr_2/1
  MATLAB Function1/14(imm32) -> imm32/1
  MATLAB Function1/18(read_en_2) -> read_en_2/1
  MATLAB Function1/15(read_addr_1) -> read_addr_1/1
  MATLAB Function1/19(write_en) -> write_en/1
  MATLAB Function1/20(alu_op) -> alu_op/1
  MATLAB Function1/21(alu_src_b) -> alu_src_b/1
  MATLAB Function1/8(ra) -> ra/1
  MATLAB Function1/9(ra_valid) -> ra_valid/1
  MATLAB Function1/10(rd_lo) -> rd_lo/1
  MATLAB Function1/11(rd_hi) -> rd_hi/1
  MATLAB Function1/12(two_wb) -> two_wb/1

== system Three_Stages/Subsystem21/Subsystem ==
  rst_n : Inport
  stall : Inport  Port=2
  data_1_in : Inport  Port=3  OutDataTypeStr=uint32
  Constant : Constant  Value=0  OutDataTypeStr=uint32
  Resettable Delay : Delay  DelayLength=1  InitialConditionSource=Input port  ExternalReset=Falling
      settings: InputPortMap=u0,r5,p4
  Switch : Switch  Criteria=u2 ~= 0  SaturateOnIntegerOverflow=off  InputSameDT=off
  data_1_out : Outport
  wires:
  data_1_in/1 -> Switch/3
  Resettable Delay/1 -> data_1_out/1, Switch/1
  Switch/1 -> Resettable Delay/1
  rst_n/1 -> Resettable Delay/2
  Constant/1 -> Resettable Delay/3
  stall/1 -> Switch/2

== system Three_Stages/Subsystem21/Subsystem1 ==
  rst_n : Inport
  stall : Inport  Port=2
  data_2_in : Inport  Port=3
  Constant : Constant  Value=0  OutDataTypeStr=uint32
  Resettable Delay : Delay  DelayLength=1  InitialConditionSource=Input port  ExternalReset=Falling
      settings: InputPortMap=u0,r5,p4
  Switch : Switch  Criteria=u2 ~= 0  OutDataTypeStr=uint32  SaturateOnIntegerOverflow=off  InputSameDT=off
  data_2_out : Outport  OutDataTypeStr=uint32
  wires:
  data_2_in/1 -> Switch/3
  Resettable Delay/1 -> data_2_out/1, Switch/1
  Switch/1 -> Resettable Delay/1
  rst_n/1 -> Resettable Delay/2
  Constant/1 -> Resettable Delay/3
  stall/1 -> Switch/2

== system Three_Stages/Subsystem21/Subsystem11 ==
  rst_n : Inport
  stall : Inport  Port=2
  alu_shamt_in : Inport  Port=3
  Constant : Constant  Value=0  OutDataTypeStr=uint8
  Resettable Delay : Delay  DelayLength=1  InitialConditionSource=Input port  ExternalReset=Falling
      settings: InputPortMap=u0,r5,p4
  Switch : Switch  Criteria=u2 ~= 0  SaturateOnIntegerOverflow=off  InputSameDT=off
  alu_shamt_out : Outport
  wires:
  alu_shamt_in/1 -> Switch/3
  Resettable Delay/1 -> alu_shamt_out/1, Switch/1
  Switch/1 -> Resettable Delay/1
  rst_n/1 -> Resettable Delay/2
  Constant/1 -> Resettable Delay/3
  stall/1 -> Switch/2

== system Three_Stages/Subsystem21/Subsystem12 ==
  rst_n : Inport
  stall : Inport  Port=2
  alu_shift_type_in : Inport  Port=3
  Constant : Constant  Value=0  OutDataTypeStr=uint8
  Resettable Delay : Delay  DelayLength=1  InitialConditionSource=Input port  ExternalReset=Falling
      settings: InputPortMap=u0,r5,p4
  Switch : Switch  Criteria=u2 ~= 0  SaturateOnIntegerOverflow=off  InputSameDT=off
  alu_shift_type_out : Outport
  wires:
  alu_shift_type_in/1 -> Switch/3
  Resettable Delay/1 -> alu_shift_type_out/1, Switch/1
  Switch/1 -> Resettable Delay/1
  rst_n/1 -> Resettable Delay/2
  Constant/1 -> Resettable Delay/3
  stall/1 -> Switch/2

== system Three_Stages/Subsystem21/Subsystem13 ==
  rst_n : Inport
  stall : Inport  Port=2
  link_pc_in : Inport  Port=3
  Constant : Constant  Value=0  OutDataTypeStr=uint32
  Resettable Delay : Delay  DelayLength=1  InitialConditionSource=Input port  ExternalReset=Falling
      settings: InputPortMap=u0,r5,p4
  Switch : Switch  Criteria=u2 ~= 0  SaturateOnIntegerOverflow=off  InputSameDT=off
  link_pc_out : Outport
  wires:
  link_pc_in/1 -> Switch/3
  Resettable Delay/1 -> link_pc_out/1, Switch/1
  Switch/1 -> Resettable Delay/1
  rst_n/1 -> Resettable Delay/2
  Constant/1 -> Resettable Delay/3
  stall/1 -> Switch/2

== system Three_Stages/Subsystem21/Subsystem14 ==
  rst_n : Inport
  stall : Inport  Port=2
  flush : Inport  Port=3
  WB_en_in : Inport  Port=4
  Constant : Constant  Value=0  OutDataTypeStr=boolean
  Constant1 : Constant  Value=0  OutDataTypeStr=uint32
  Resettable Delay : Delay  DelayLength=1  InitialConditionSource=Input port  ExternalReset=Falling
      settings: InputPortMap=u0,r5,p4
  Switch : Switch  Criteria=u2 ~= 0  OutDataTypeStr=boolean  SaturateOnIntegerOverflow=off  InputSameDT=off
  Switch1 : Switch  Criteria=u2 ~= 0  OutDataTypeStr=boolean  SaturateOnIntegerOverflow=off  InputSameDT=off
  WB_en_out : Outport
  wires:
  Constant1/1 -> Switch1/1
  Switch1/1 -> Resettable Delay/1
  Resettable Delay/1 -> WB_en_out/1, Switch/1
  Constant/1 -> Resettable Delay/3
  flush/1 -> Switch1/2
  rst_n/1 -> Resettable Delay/2
  Switch/1 -> Switch1/3
  stall/1 -> Switch/2
  WB_en_in/1 -> Switch/3

== system Three_Stages/Subsystem21/Subsystem15 ==
  rst_n : Inport
  stall : Inport  Port=2
  flush : Inport  Port=3
  opcode_in : Inport  Port=4
  Constant : Constant  Value=127  OutDataTypeStr=uint8
  Constant1 : Constant  Value=127  OutDataTypeStr=uint8
  Resettable Delay : Delay  DelayLength=1  InitialConditionSource=Input port  ExternalReset=Falling
      settings: InputPortMap=u0,r5,p4
  Switch : Switch  Criteria=u2 ~= 0  SaturateOnIntegerOverflow=off  InputSameDT=off
  Switch1 : Switch  Criteria=u2 ~= 0  SaturateOnIntegerOverflow=off  InputSameDT=off
  opcode_out : Outport
  wires:
  Constant1/1 -> Switch1/1
  Switch1/1 -> Resettable Delay/1
  Resettable Delay/1 -> opcode_out/1, Switch/1
  Constant/1 -> Resettable Delay/3
  flush/1 -> Switch1/2
  rst_n/1 -> Resettable Delay/2
  Switch/1 -> Switch1/3
  stall/1 -> Switch/2
  opcode_in/1 -> Switch/3

== system Three_Stages/Subsystem21/Subsystem16 ==
  rst_n : Inport
  stall : Inport  Port=2
  flush : Inport  Port=3
  cond_in : Inport  Port=4
  Constant : Constant  Value=0  OutDataTypeStr=uint8
  Constant1 : Constant  Value=0  OutDataTypeStr=uint8
  Resettable Delay : Delay  DelayLength=1  InitialConditionSource=Input port  ExternalReset=Falling
      settings: InputPortMap=u0,r5,p4
  Switch : Switch  Criteria=u2 ~= 0  OutDataTypeStr=uint8  SaturateOnIntegerOverflow=off  InputSameDT=off
  Switch1 : Switch  Criteria=u2 ~= 0  OutDataTypeStr=uint8  SaturateOnIntegerOverflow=off  InputSameDT=off
  cond_out : Outport
  wires:
  Constant1/1 -> Switch1/1
  Switch1/1 -> Resettable Delay/1
  Resettable Delay/1 -> cond_out/1, Switch/1
  Constant/1 -> Resettable Delay/3
  flush/1 -> Switch1/2
  rst_n/1 -> Resettable Delay/2
  Switch/1 -> Switch1/3
  stall/1 -> Switch/2
  cond_in/1 -> Switch/3
